simulink model "three_boards_receiver"  (R2025a)
settings: Solver=FixedStepDiscrete  StartTime=0.0  StopTime=inf  FixedStep=Ts  MaxStep=Ts  RelTol=1e-3
model workspace (MAT data in the model file):
  Ts = Simulink.Parameter
  Ts.Value = 0.1
  Ts.DataType = 'auto'
  Ts.Complexity = 'real'
  Ts.Dimensions = [1 1]
undefined symbols (not defined in the file): CAN_ANGLE_ICUB2DEG, canChannel
libraries: canmsglib x7, hdlsllib x3, canlib x2, dspswit3 x1, sldrtlib x1
settings Model: DataDictionary=EmbeddedBoardDD.sldd  SimulationMode=accelerator  Creator=mfussi  LastModifiedBy=mfussi
settings SolverCC: AutoInsertRateTranBlk=on
settings OptimizationCC: SimCompilerOptimization=on
settings ModelReferenceCC: UpdateModelReferenceTargets=Force
settings SFSimCC: SimHardwareAcceleration=native
settings RTWCC: BuildConfiguration=Faster Runs  GPUComputeCapability=3.5

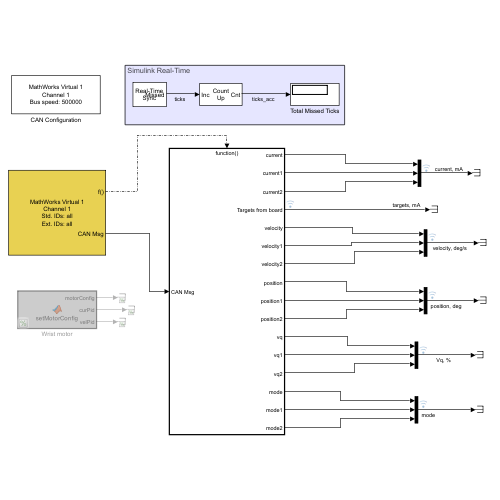
[thumbnail: Simulink's stored preview of the top-level diagram]
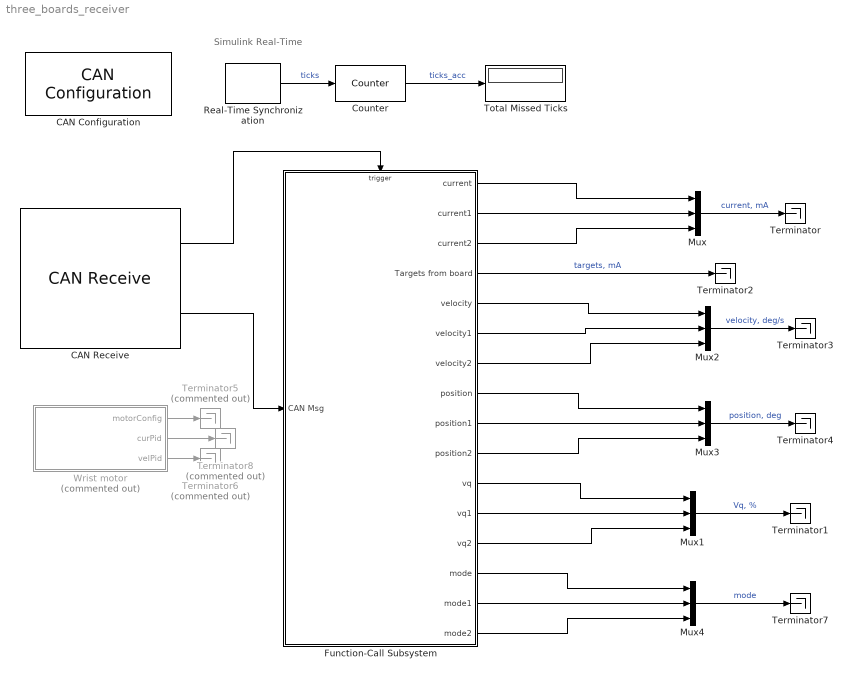
== system three_boards_receiver ==
  note: Simulink Real-Time
  CAN Configuration : canlib/CAN Configuration  BlockHandle=241105.0015  Device=MathWorks Virtual 1 (Channel 1)  DeviceMenu=MathWorks Virtual 1 (Channel 1)  ObjConstructor=canChannel('MathWorks', 'Virtual 1', 1)  BusSpeed=500000  EnableBitParameters=off  AckMode=Normal
  CAN Receive : canlib/CAN Receive  BlockHandle=3.0037  Device=MathWorks Virtual 1 (Channel 1)  DeviceMenu=MathWorks Virtual 1 (Channel 1)  ObjConstructor=canChannel('MathWorks', 'Virtual 1', 1)  EnableStandardIDsFilter=off  StdIDsCombo=Allow all  StandardIDs=0  EnableExtendedIDsFilter=off  ExtIDsCombo=Allow all  ExtendedIDs=0  SampleTime=Ts  MsgsPerTimestep=all  InternalFilterUpdateStatus=on  BusOutput=on
  Counter : dspswit3/Counter  Direction=Up  CountEvent=Rising edge  CounterSize=32 bits  MaxCount=255  InitialCount=0  Output=Count  HitValue=32  ResetInput=off  SamplesPerFrame=1  Ts=1  CntDtype=uint32  HitDtype=Logical
  Function-Call Subsystem : Subsystem  TreatAsAtomicUnit=on
  Mux{,1..4} (5 alike) : Mux  Inputs=3
  Real-Time Synchronization : sldrtlib/Real-Time Synchronization  SampleTime=Ts  MaxMissedTicks=inf  ShowMissedTicks=on  YieldWhenWaiting=off
  Terminator{,1..4,7} (6 alike) : Terminator
  Terminator5 : Terminator  Commented=on
  Terminator6 : Terminator  Commented=on
  Terminator8 : Terminator  Commented=on
  Total Missed Ticks : Display
      settings: Decimation=5
  Wrist motor : MATLAB Function  Commented=on  TreatAsAtomicUnit=on
  wires:
  Real-Time Synchronization/1 -> Counter/1  "ticks"
  Counter/1 -> Total Missed Ticks/1  "ticks_acc"
  Function-Call Subsystem/4(Targets from board) -> Terminator2/1  "targets, mA"
  CAN Receive/2 -> Function-Call Subsystem/1(CAN Msg)
  CAN Receive/1 -> Function-Call Subsystem/Trigger
  Function-Call Subsystem/1(current) -> Mux/1
  Function-Call Subsystem/3(current2) -> Mux/3
  Function-Call Subsystem/2(current1) -> Mux/2
  Function-Call Subsystem/11(vq) -> Mux1/1
  Function-Call Subsystem/12(vq1) -> Mux1/2
  Function-Call Subsystem/13(vq2) -> Mux1/3
  Mux/1 -> Terminator/1  "current, mA"
  Mux1/1 -> Terminator1/1  "Vq, %"
  Mux2/1 -> Terminator3/1  "velocity, deg/s"
  Function-Call Subsystem/5(velocity) -> Mux2/1
  Function-Call Subsystem/6(velocity1) -> Mux2/2
  Function-Call Subsystem/7(velocity2) -> Mux2/3
  Function-Call Subsystem/8(position) -> Mux3/1
  Function-Call Subsystem/9(position1) -> Mux3/2
  Function-Call Subsystem/10(position2) -> Mux3/3
  Mux3/1 -> Terminator4/1  "position, deg"
  Wrist motor/1(motorConfig) -> Terminator5/1
  Wrist motor/3(velPid) -> Terminator6/1
  Function-Call Subsystem/14(mode) -> Mux4/1
  Function-Call Subsystem/15(mode1) -> Mux4/2
  Function-Call Subsystem/16(mode2) -> Mux4/3
  Mux4/1 -> Terminator7/1  "mode"
  Wrist motor/2(curPid) -> Terminator8/1

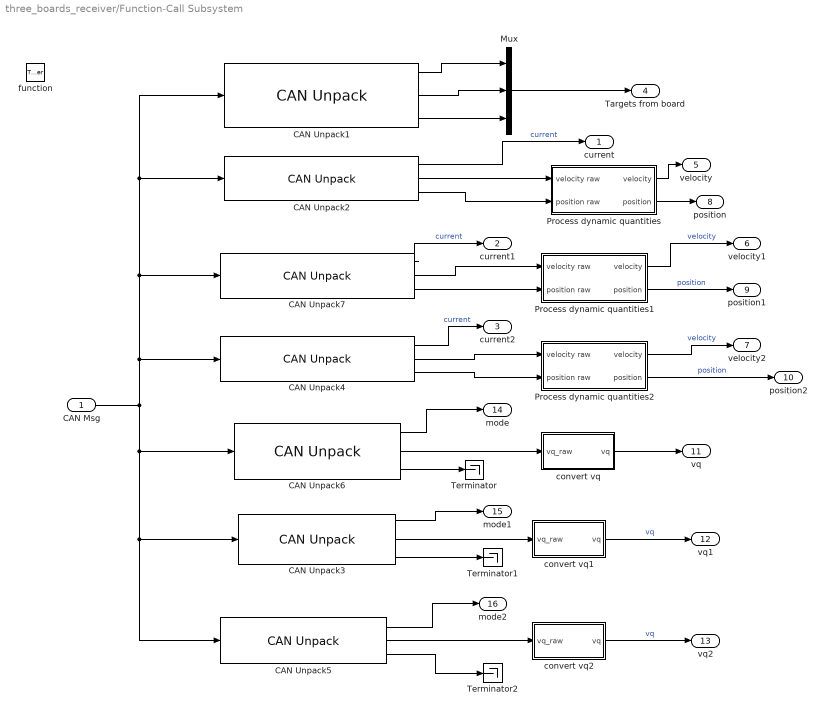
== system three_boards_receiver/Function-Call Subsystem ==
  CAN Msg : Inport
  function : TriggerPort  TriggerType=function-call  VariantControl=(inherit)
  CAN Unpack1 : canmsglib/CAN Unpack  MsgList=(none)  MsgName=TARGETS  MsgIDType=Standard (11-bit identifier)  MsgIdentifier=0x10F  MsgLength=8  SignalInfo={ 'Target1', '0', '16', 'LE', 'signed', 'Standard', '0', '1', '0', '-Inf', 'Inf'; 'Target2', '16', '16', 'LE', 'signed', 'Standard', '0', '1', '0', '-Inf', 'Inf'; 'Target3', '32', '16', 'LE', 'signed', 'Standard', '0', '1', '0', '-Inf', 'Inf' }  IDPort=off  TimestampPort=off  ErrorPort=off  RemotePort=off  LengthPort=off  StatusPort=off  ApplyMinMax=off
  CAN Unpack2 : canmsglib/CAN Unpack  MsgList=(none)  MsgName=FOC  MsgIDType=Standard (11-bit identifier)  MsgIdentifier=0x110  MsgLength=8  SignalInfo={ 'current', '0', '16', 'LE', 'signed', 'Standard', '0', '1', '0', '-Inf', 'Inf'; 'velocity', '16', '16', 'LE', 'signed', 'Standard', '0', '1', '0', '-Inf', 'Inf'; 'position', '32', '32', 'LE', 'signed', 'Standard', '0', '1', '0', '-Inf', 'Inf' }  IDPort=off  TimestampPort=off  ErrorPort=off  RemotePort=off  LengthPort=off  StatusPort=off  ApplyMinMax=off
  CAN Unpack3 : canmsglib/CAN Unpack  MsgList=(none)  MsgName=STATUS  MsgIDType=Standard (11-bit identifier)  MsgIdentifier=0x123  MsgLength=8  SignalInfo={ 'mode', '0', '8', 'LE', 'unsigned', 'Standard', '0', '1', '0', '-Inf', 'Inf'; 'pwm', '16', '16', 'LE', 'signed', 'Standard', '0', '1', '0', '-Inf', 'Inf'; 'fault', '32', '8', 'LE', 'unsigned', 'Standard', '0', '1', '0', '-Inf', 'Inf' }  IDPort=off  TimestampPort=off  ErrorPort=off  RemotePort=off  LengthPort=off  StatusPort=off  ApplyMinMax=off
  CAN Unpack4 : canmsglib/CAN Unpack  MsgList=(none)  MsgName=FOC  MsgIDType=Standard (11-bit identifier)  MsgIdentifier=0x130  MsgLength=8  SignalInfo={ 'current', '0', '16', 'LE', 'signed', 'Standard', '0', '1', '0', '-Inf', 'Inf'; 'velocity', '16', '16', 'LE', 'signed', 'Standard', '0', '1', '0', '-Inf', 'Inf'; 'position', '32', '32', 'LE', 'signed', 'Standard', '0', '1', '0', '-Inf', 'Inf' }  IDPort=off  TimestampPort=off  ErrorPort=off  RemotePort=off  LengthPort=off  StatusPort=off  ApplyMinMax=off
  CAN Unpack5 : canmsglib/CAN Unpack  MsgList=(none)  MsgName=STATUS  MsgIDType=Standard (11-bit identifier)  MsgIdentifier=0x133  MsgLength=8  SignalInfo={ 'mode', '0', '8', 'LE', 'unsigned', 'Standard', '0', '1', '0', '-Inf', 'Inf'; 'pwm', '16', '16', 'LE', 'signed', 'Standard', '0', '1', '0', '-Inf', 'Inf'; 'fault', '32', '8', 'LE', 'unsigned', 'Standard', '0', '1', '0', '-Inf', 'Inf' }  IDPort=off  TimestampPort=off  ErrorPort=off  RemotePort=off  LengthPort=off  StatusPort=off  ApplyMinMax=off
  CAN Unpack6 : canmsglib/CAN Unpack  MsgList=(none)  MsgName=STATUS  MsgIDType=Standard (11-bit identifier)  MsgIdentifier=0x113  MsgLength=8  SignalInfo={ 'mode', '0', '8', 'LE', 'unsigned', 'Standard', '0', '1', '0', '-Inf', 'Inf'; 'pwm', '16', '16', 'LE', 'signed', 'Standard', '0', '1', '0', '-Inf', 'Inf'; 'fault', '32', '8', 'LE', 'unsigned', 'Standard', '0', '1', '0', '-Inf', 'Inf' }  IDPort=off  TimestampPort=off  ErrorPort=off  RemotePort=off  LengthPort=off  StatusPort=off  ApplyMinMax=off
  CAN Unpack7 : canmsglib/CAN Unpack  MsgList=(none)  MsgName=FOC  MsgIDType=Standard (11-bit identifier)  MsgIdentifier=0x120  MsgLength=8  SignalInfo={ 'current', '0', '16', 'LE', 'signed', 'Standard', '0', '1', '0', '-Inf', 'Inf'; 'velocity', '16', '16', 'LE', 'signed', 'Standard', '0', '1', '0', '-Inf', 'Inf'; 'position', '32', '32', 'LE', 'signed', 'Standard', '0', '1', '0', '-Inf', 'Inf' }  IDPort=off  TimestampPort=off  ErrorPort=off  RemotePort=off  LengthPort=off  StatusPort=off  ApplyMinMax=off
  Mux : Mux  Inputs=3
  Process dynamic quantities : Subsystem
  Process dynamic quantities1 : Subsystem
  Process dynamic quantities2 : Subsystem
  Terminator : Terminator
  Terminator1 : Terminator
  Terminator2 : Terminator
  convert vq : Subsystem
  convert vq1 : Subsystem
  convert vq2 : Subsystem
  current : Outport  Unit=mA
  current1 : Outport  Port=2  Unit=mA
  current2 : Outport  Port=3  Unit=mA
  Targets from board : Outport  Port=4
  velocity : Outport  Port=5
  velocity1 : Outport  Port=6
  velocity2 : Outport  Port=7
  position : Outport  Port=8
  position1 : Outport  Port=9
  position2 : Outport  Port=10
  vq : Outport  Port=11  PortDimensions=1
  vq1 : Outport  Port=12  PortDimensions=1
  vq2 : Outport  Port=13  PortDimensions=1
  mode : Outport  Port=14
  mode1 : Outport  Port=15
  mode2 : Outport  Port=16
  wires:
  CAN Unpack2/1 -> current/1  "current"
  CAN Unpack1/1 -> Mux/1
  CAN Unpack1/2 -> Mux/2
  CAN Unpack1/3 -> Mux/3
  Mux/1 -> Targets from board/1
  Process dynamic quantities1/1(velocity) -> velocity1/1  "velocity"
  CAN Unpack7/1 -> current1/1  "current"
  Process dynamic quantities1/2(position) -> position1/1  "position"
  CAN Msg/1 -> CAN Unpack4/1, CAN Unpack1/1, CAN Unpack2/1, CAN Unpack7/1, CAN Unpack5/1, CAN Unpack3/1, CAN Unpack6/1
  Process dynamic quantities2/1(velocity) -> velocity2/1  "velocity"
  Process dynamic quantities2/2(position) -> position2/1  "position"
  CAN Unpack4/1 -> current2/1  "current"
  CAN Unpack2/2 -> Process dynamic quantities/1(velocity raw)
  CAN Unpack2/3 -> Process dynamic quantities/2(position raw)
  Process dynamic quantities/1(velocity) -> velocity/1
  Process dynamic quantities/2(position) -> position/1
  CAN Unpack7/2 -> Process dynamic quantities1/1(velocity raw)
  CAN Unpack7/3 -> Process dynamic quantities1/2(position raw)
  CAN Unpack4/2 -> Process dynamic quantities2/1(velocity raw)
  CAN Unpack4/3 -> Process dynamic quantities2/2(position raw)
  CAN Unpack6/1 -> mode/1
  CAN Unpack3/2 -> convert vq1/1(vq_raw)
  convert vq1/1(vq) -> vq1/1  "vq"
  CAN Unpack5/2 -> convert vq2/1(vq_raw)
  convert vq2/1(vq) -> vq2/1  "vq"
  CAN Unpack3/1 -> mode1/1
  CAN Unpack5/1 -> mode2/1
  CAN Unpack6/2 -> convert vq/1(vq_raw)
  convert vq/1(vq) -> vq/1
  CAN Unpack6/3 -> Terminator/1
  CAN Unpack3/3 -> Terminator1/1
  CAN Unpack5/3 -> Terminator2/1

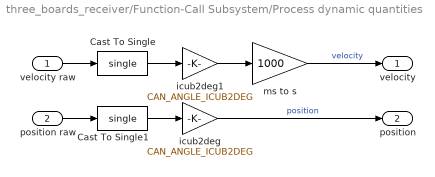
== system three_boards_receiver/Function-Call Subsystem/Process dynamic quantities ==
  velocity raw : Inport
  position raw : Inport  Port=2
  Cast To Single : DataTypeConversion  OutDataTypeStr=single  SaturateOnIntegerOverflow=off  RndMeth=Floor
  Cast To Single1 : DataTypeConversion  OutDataTypeStr=single  SaturateOnIntegerOverflow=off  RndMeth=Floor
  icub2deg : Gain  Gain=CAN_ANGLE_ICUB2DEG
  icub2deg1 : Gain  Gain=CAN_ANGLE_ICUB2DEG
  ms to s : Gain  Gain=1000
  velocity : Outport
  position : Outport  Port=2
  wires:
  Cast To Single1/1 -> icub2deg/1
  icub2deg1/1 -> ms to s/1
  Cast To Single/1 -> icub2deg1/1
  icub2deg/1 -> position/1  "position"
  velocity raw/1 -> Cast To Single/1
  position raw/1 -> Cast To Single1/1
  ms to s/1 -> velocity/1  "velocity"

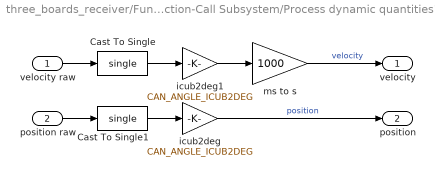
== system three_boards_receiver/Function-Call Subsystem/Process dynamic quantities1 ==
  velocity raw : Inport
  position raw : Inport  Port=2
  Cast To Single : DataTypeConversion  OutDataTypeStr=single  SaturateOnIntegerOverflow=off  RndMeth=Floor
  Cast To Single1 : DataTypeConversion  OutDataTypeStr=single  SaturateOnIntegerOverflow=off  RndMeth=Floor
  icub2deg : Gain  Gain=CAN_ANGLE_ICUB2DEG
  icub2deg1 : Gain  Gain=CAN_ANGLE_ICUB2DEG
  ms to s : Gain  Gain=1000
  velocity : Outport
  position : Outport  Port=2
  wires:
  Cast To Single1/1 -> icub2deg/1
  icub2deg1/1 -> ms to s/1
  Cast To Single/1 -> icub2deg1/1
  icub2deg/1 -> position/1  "position"
  velocity raw/1 -> Cast To Single/1
  position raw/1 -> Cast To Single1/1
  ms to s/1 -> velocity/1  "velocity"

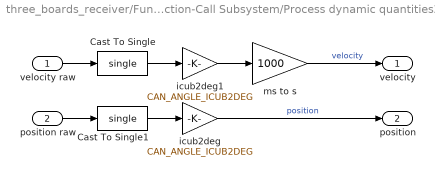
== system three_boards_receiver/Function-Call Subsystem/Process dynamic quantities2 ==
  velocity raw : Inport
  position raw : Inport  Port=2
  Cast To Single : DataTypeConversion  OutDataTypeStr=single  SaturateOnIntegerOverflow=off  RndMeth=Floor
  Cast To Single1 : DataTypeConversion  OutDataTypeStr=single  SaturateOnIntegerOverflow=off  RndMeth=Floor
  icub2deg : Gain  Gain=CAN_ANGLE_ICUB2DEG
  icub2deg1 : Gain  Gain=CAN_ANGLE_ICUB2DEG
  ms to s : Gain  Gain=1000
  velocity : Outport
  position : Outport  Port=2
  wires:
  Cast To Single1/1 -> icub2deg/1
  icub2deg1/1 -> ms to s/1
  Cast To Single/1 -> icub2deg1/1
  icub2deg/1 -> position/1  "position"
  velocity raw/1 -> Cast To Single/1
  position raw/1 -> Cast To Single1/1
  ms to s/1 -> velocity/1  "velocity"

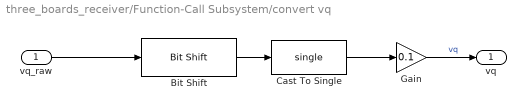
== system three_boards_receiver/Function-Call Subsystem/convert vq ==
  vq_raw : Inport
  Bit Shift : hdlsllib/Logic and Bit Operations/Bit Shift  mode=Shift Left Logical  N=1
  Cast To Single : DataTypeConversion  OutDataTypeStr=single  SaturateOnIntegerOverflow=off  RndMeth=Floor
  Gain : Gain  Gain=0.1
  vq : Outport
  wires:
  Bit Shift/1 -> Cast To Single/1
  vq_raw/1 -> Bit Shift/1
  Cast To Single/1 -> Gain/1
  Gain/1 -> vq/1  "vq"

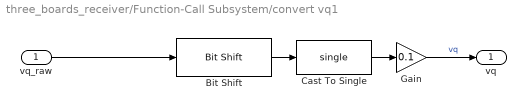
== system three_boards_receiver/Function-Call Subsystem/convert vq1 ==
  vq_raw : Inport
  Bit Shift : hdlsllib/Logic and Bit Operations/Bit Shift  mode=Shift Left Logical  N=1
  Cast To Single : DataTypeConversion  OutDataTypeStr=single  SaturateOnIntegerOverflow=off  RndMeth=Floor
  Gain : Gain  Gain=0.1
  vq : Outport
  wires:
  Bit Shift/1 -> Cast To Single/1
  vq_raw/1 -> Bit Shift/1
  Cast To Single/1 -> Gain/1
  Gain/1 -> vq/1  "vq"

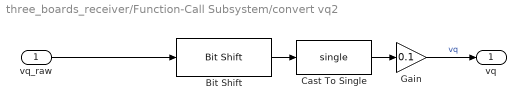
== system three_boards_receiver/Function-Call Subsystem/convert vq2 ==
  vq_raw : Inport
  Bit Shift : hdlsllib/Logic and Bit Operations/Bit Shift  mode=Shift Left Logical  N=1
  Cast To Single : DataTypeConversion  OutDataTypeStr=single  SaturateOnIntegerOverflow=off  RndMeth=Floor
  Gain : Gain  Gain=0.1
  vq : Outport
  wires:
  Bit Shift/1 -> Cast To Single/1
  vq_raw/1 -> Bit Shift/1
  Cast To Single/1 -> Gain/1
  Gain/1 -> vq/1  "vq"

== matlab function three_boards_receiver/Wrist motor ==
  data: motorConfig output Bus: MotorConfig; curPid output Bus: PIDConfig; velPid output Bus: PIDConfig
function [motorConfig, curPid, velPid] = setMotorConfig()

motorConfig.has_hall_sens = true;
motorConfig.has_quadrature_encoder = false;
motorConfig.has_speed_quadrature_encoder = false;
motorConfig.has_torque_sens = false;
motorConfig.use_index = false;
motorConfig.enable_verbosity = true;
motorConfig.rotor_encoder_resolution = int16(0); % set to 0 to use only hall sensors
motorConfig.rotor_index_offset = int16(0);
motorConfig.encoder_tolerance = uint8(0);
motorConfig.pole_pairs = uint8(7);
motorConfig.Kbemf = single(0);
motorConfig.Rphase = single(0);
motorConfig.Imin = single(-1e3);
motorConfig.Imax = single(1e3);
motorConfig.Vcc = single(24);
motorConfig.Vmax = single(24);

% Hall offset and BC phases swap is not available as a CAN message
% The parameters need to be changed in rtw_motor_config.c
hall_offset = 120; % degrees
swap_bc = 1;

% ---------------------------------

curPid.OutMax = single(100);
curPid.OutMin = single(-100);
curPid.P = single(2);
curPid.I = single(500);
curPid.D = single(0);
curPid.N = single(100);
curPid.I0 = single(0);
curPid.D0 = single(0);
curPid.shift_factor = uint8(6);


velPid.OutMax = single(1000);
velPid.OutMin = single(-1000);
velPid.P = single(-1000);
velPid.I = single(-1000);
velPid.D = single(0);
velPid.N = single(100);
velPid.I0 = single(0);
velPid.D0 = single(0);
velPid.shift_factor = uint8(10);
